simulink model "three_phase_rl_load"  (R2026b)
settings: Solver=VariableStepAuto
libraries: fl_lib x3
settings Model: Creator=ltnbda  LastModifiedBy=d.bagnara
settings RTWCC: GPUComputeCapability=5.0

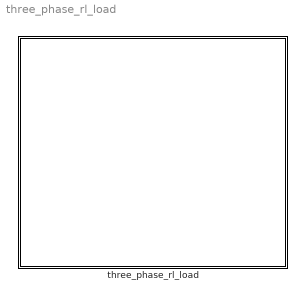
== system three_phase_rl_load ==
  three_phase_rl_load : Subsystem  mask{Ls1_load_m=1e-3, Rs1_load_m=1, Ls2_load_m=1e-3, Rs2_load_m=1, Ls3_load_m=1e-3, Rs3_load_m=1}
      mask prompts: Ls1_load_m "Ls1_load (H)"; Rs1_load_m "Rs1_load (Ohm)"; Ls2_load_m "Ls2_load (H)"; Rs2_load_m "Rs2_load (Ohm)"; Ls3_load_m "Ls3_load (H)"; Rs3_load_m "Rs3_load (Ohm)"
      mask Display:
      | disp('Three Phase RL Load');
      | port_label('lconn', 1, 'u1');
      | port_label('lconn', 2, 'v1');
      | port_label('lconn', 3, 'w1');

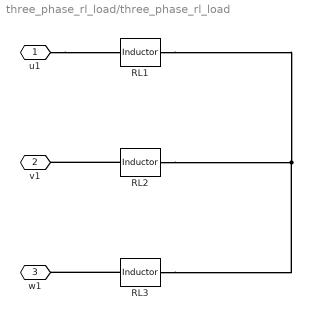
== system three_phase_rl_load/three_phase_rl_load ==
  RL1 : fl_lib/Electrical/Electrical Elements/Inductor  l=Ls1_load_m H  r=Rs1_load_m Ohm  g=1e-9 1/Ohm  i_specify=off  i_priority=None  i=0 A  i_nominal_specify=off  i_nominal_value=1  i_nominal_unit=A  v_specify=off  v_priority=None  v=0 V  v_nominal_specify=off  v_nominal_value=1  v_nominal_unit=V  i_L_specify=off  i_L_priority=High  i_L=0 A  i_L_nominal_specify=off  i_L_nominal_value=1  i_L_nominal_unit=A
  RL2 : fl_lib/Electrical/Electrical Elements/Inductor  l=Ls2_load_m H  r=Rs2_load_m Ohm  g=1e-9 1/Ohm  i_specify=off  i_priority=None  i=0 A  i_nominal_specify=off  i_nominal_value=1  i_nominal_unit=A  v_specify=off  v_priority=None  v=0 V  v_nominal_specify=off  v_nominal_value=1  v_nominal_unit=V  i_L_specify=off  i_L_priority=High  i_L=0 A  i_L_nominal_specify=off  i_L_nominal_value=1  i_L_nominal_unit=A
  RL3 : fl_lib/Electrical/Electrical Elements/Inductor  l=Ls3_load_m H  r=Rs3_load_m Ohm  g=1e-9 1/Ohm  i_specify=off  i_priority=None  i=0 A  i_nominal_specify=off  i_nominal_value=1  i_nominal_unit=A  v_specify=off  v_priority=None  v=0 V  v_nominal_specify=off  v_nominal_value=1  v_nominal_unit=V  i_L_specify=off  i_L_priority=High  i_L=0 A  i_L_nominal_specify=off  i_L_nominal_value=1  i_L_nominal_unit=A
  u1 : PMIOPort  Side=Left
  v1 : PMIOPort  Port=2  Side=Left
  w1 : PMIOPort  Port=3  Side=Left
  connections:
  u1/RConn1 -- RL1/LConn1
  RL3/LConn1 -- w1/RConn1
  RL2/LConn1 -- v1/RConn1
  RL1/RConn1 -- RL3/RConn1 -- RL2/RConn1
